simulink model "RM3"  (R2020b)
settings: Solver=ode4  StartTime=0  StopTime=400  FixedStep=0.1  MaxStep=0.1  RelTol=1e-3  EnableMultiTasking=on
undefined symbols (not defined in the file or in its folder): body, constraint, geometry, hydroData, pto
libraries: WECSim_Lib_Body_Elements x2, WECSim_Lib_Constraints x1, WECSim_Lib_Frames x1, WECSim_Lib_PTOs x1
settings Model: Creator=mlawson  LastModifiedBy=akeeste
settings SolverCC: ZeroCrossControl=DisableAll  AlgebraicLoopSolver=LineSearch  AutoInsertRateTranBlk=on
settings DataIOCC: SaveFormat=Array  SaveOutput=off  SaveTime=off  ReturnWorkspaceOutputs=off
settings OptimizationCC: LifeSpan=inf  SimCompilerOptimization=on
settings DebuggingCC: UnderspecifiedInitializationDetection=Classic  MergeDetectMultiDrivingBlocksExec=none  SolverPrmCheckMsg=warning  AllowSymbolicDim=off  StateNameClashWarn=warning  SFUnexpectedBacktrackingDiag=warning  SFNoUnconditionalDefaultTransitionDiag=warning  SFExecutionAtInitializationDiag=none  ArithmeticOperatorsInVariantConditions=warning
settings HardwareCC: ProdBitPerPointer=32  ProdBitPerSizeT=32  ProdBitPerPtrDiffT=32  ProdLargestAtomicFloat=None  ProdIntDivRoundTo=Undefined  ProdEndianess=Unspecified  ProdWordSize=32  ProdHWDeviceType=32-bit Generic
settings ModelReferenceCC: PropagateSignalLabelsOutOfModel=off
settings SFSimCC: SimUseLocalCustomCode=off  CustomCodeUndefinedFunction=UseInterfaceOnly
settings RTWCC: RTWUseLocalCustomCode=off
settings CodeAppCC: StateflowObjectComments=on
settings GRTTargetCC: TargetLangStandard=C89/C90 (ANSI)
settings ConfigComp: CovMetricSettings=dw  CovSaveCumulativeToWorkspaceVar=on  CovSaveSingleToWorkspaceVar=on  CovExternalEMLEnable=off  CovSFcnEnable=off
settings SimscapeCC: SimscapeNormalizeSystem=off
settings ConfigurationSet: Description=SimMechanics 2G
settings ExplorerConfigSet: InternalSimMechanicsExplorerSettings="<ExplorerConfiguration><canonicalview>default</canonicalview><AnimationSetting><BasePlaybackSpeed>1.0</BasePlaybackSpeed><PlaybackSpeedFactor>1.0</PlaybackSpeedFactor></AnimationSetting><TilePanel><TileInfo><Tiles Columns=\"2\" Count=\"4\" Rows=\"2\"><Column Weight=\"0.5\"/><Column Weight=\"0.5\"/><Row Weight=\"0.5\"/><Row Weight=\"0.5\"/><Tile Height=\"1\" Width=\"1\" X=\"0\" Y=\"0\"/><Tile Height=\"1\" Width=\"1\" X=\"0\" Y=\"1\"/><Tile Height=\"1\" Width=\"1\" X=\"1\" Y=\"0\"/><Tile Height=\"1\" Width=\"1\" X=\"1\" Y=\"1\"/></Tiles></TileInfo><SceneInfo><SceneViewer><BGColor><R>0.60000002384185791</R><G>0.60000002384185791</G><B>0.60000002384185791</B></BGColor><Camera><DoPerspective>off</DoPerspective><Position><X>-5.28910957848137908</X><Y>-384.632249072613831</Y><Z>-15.1490561438029978</Z></Position><Center><X>-5.28910957848137908</X><Y>-7.28939721739152446e-06</Y><Z>-15.1490561438029978</Z></Center><Up><X>0</X><Y>-0</Y><Z>1</Z></Up><ViewLimDist>1</ViewLimDist><YLim>29.7178180022969975</YLim><XLim>34.354994301313134</XLim></Camera></SceneViewer><SceneViewer><BGColor><R>0.60000002384185791</R><G>0.60000002384185791</G><B>0.60000002384185791</B></BGColor><Camera><DoPerspective>off</DoPerspective><Position><X>-1.1840554071884688</X><Y>-5.46187101601080105</Y><Z>285.569034477344985</Z></Position><Center><X>-1.1840554071884688</X><Y>-5.46187101601080105</Y><Z>-96.4189878956305506</Z></Center><Up><X>0</X><Y>1</Y><Z>-0</Z></Up><ViewLimDist>1</ViewLimDist><YLim>38.1722158903479212</YLim><XLim>44.1286187054525456</XLim></Camera></SceneViewer><SceneViewer><BGColor><R>0.60000002384185791</R><G>0.60000002384185791</G><B>0.60000002384185791</B></BGColor><Camera><DoPerspective>off</DoPerspective><Position><X>384.632249217085132</X><Y>0.260362946589576594</Y><Z>-15.6955920945191423</Z></Position><Center><X>-7.15773737169911328e-06</X><Y>0.260362946589576594</Y><Z>-15.6955920945191423</Z></Center><Up><X>-0</X><Y>0</Y><Z>1</Z></Up><ViewLimDist>1</ViewLimDist><YLim>30.7766093059417472</YLim><XLim>35.5789996842178908</XLim></Camera></SceneViewer><SceneViewer><BGColor><R>0.60000002384185791</R><G>0.60000002384185791</G><B>0.60000002384185791</B></BGColor><Camera><DoPerspective>off</DoPerspective><Position><X>191.32988391583163</X><Y>-195.842532631356448</Y><Z>177.457736592884231</Z></Position><Center><X>-30.2968327101377994</X><Y>25.7841839946129028</Y><Z>-44.1689800330834714</Z></Center><Up><X>-0.408248290463863073</X><Y>0.408248290463863073</Y><Z>0.816496580927726145</Z></Up><ViewLimDist>1</ViewLimDist><YLim>34.6800041830381574</YLim><XLim>40.0914813458276669</XLim></Camera></SceneViewer></SceneInfo></TilePanel><MechEditorPanel><Cameras/><GfxPanelCameraMap/><VideoCreator><PlaybackSpeedRatio>1.0</PlaybackSpeedRatio><FrameRate>30</FrameRate><VideoFormat>Motion JPEG AVI</VideoFormat><FrameSize>auto</FrameSize></VideoCreator></MechEditorPanel></ExplorerConfiguration>"

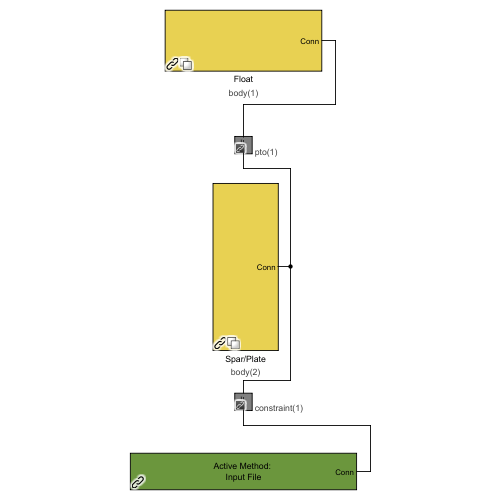
[thumbnail: Simulink's stored preview of the top-level diagram]
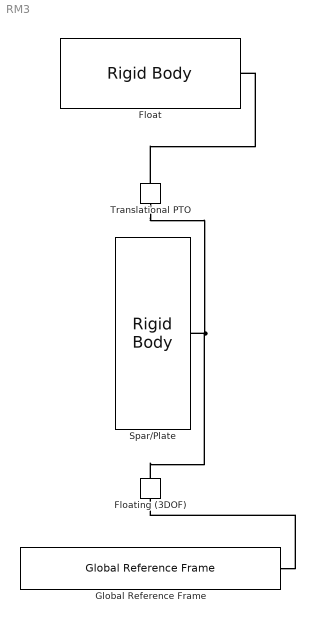
== system RM3 ==
  Float : WECSim_Lib_Body_Elements/Rigid Body  body=body(1)  h5File=hydroData/*.h5  geometryFile=geometry/*.stl  mass=0  inertia=0 0 0  inertiaProducts=0 0 0  nonHydro=0  nonlinearHydro=0  centerGravity=0 0 0  centerBuoyancy=0 0 0  dof=6  volume=0  displacement=0 0 0  axis=0 1 0  angle=0  option=0  cd=0 0 0  ca=0 0 0  area=0 0 0  VME=0  rgME=0 0 0  z=0 0 1
  Floating (3DOF) : WECSim_Lib_Constraints/Floating (3DOF)  constraint=constraint(1)  loc="0  0  0"  displacement=0 0 0  y=0 1 0  z=0 0 1  upperLimitSpecify=off  upperLimitBound=0  upperLimitTransitionRegionWidth=0  upperLimitStiffness=0  upperLimitDamping=0  lowerLimitSpecify=off  lowerLimitBound=0  lowerLimitTransitionRegionWidth=0  lowerLimitStiffness=0  lowerLimitDamping=0
      settings: AttributesFormatString=%<constraint>
  Global Reference Frame : WECSim_Lib_Frames/Global Reference Frame  waves=waves  simu=simu  InputMethod=Input File  InputFile=wecSimInputFile.m  mode=normal  explorer=off  solver=ode4  startTime=0  rampTime=100  endTime=400  dt=0.1  cicEndTime=60  stateSpace=0  WaveClass=regular  height=2.5  period=8  elevationFile=NOT DEFINED  spectrumFile=NOT DEFINED  direction=0  spread=1  spectrumType=NOT DEFINED  phaseSeed=0  option=EqualEnergy
  Spar/Plate : WECSim_Lib_Body_Elements/Rigid Body  body=body(2)  h5File=hydroData/*.h5  geometryFile=geometry/*.stl  mass=0  inertia=0 0 0  inertiaProducts=0 0 0  nonHydro=0  nonlinearHydro=0  centerGravity=0 0 0  centerBuoyancy=0 0 0  dof=6  volume=0  displacement=0 0 0  axis=0 1 0  angle=0  option=0  cd=0 0 0  ca=0 0 0  area=0 0 0  VME=0  rgME=0 0 0  z=0 0 1
  Translational PTO : WECSim_Lib_PTOs/Translational PTO  pto=pto(1)  loc="0  0  0"  stiffness=0  damping=0  equilibriumPosition=0  pretension=0  displacement=0 0 0  y=0 1 0  z=0 0 1  upperLimitSpecify=off  upperLimitBound=0  upperLimitTransitionRegionWidth=0  upperLimitStiffness=0  upperLimitDamping=0  lowerLimitSpecify=off  lowerLimitBound=0  lowerLimitTransitionRegionWidth=0  lowerLimitStiffness=0  lowerLimitDamping=0
      settings: AttributesFormatString=%<pto>
  connections:
  Global Reference Frame/RConn1 -- Floating (3DOF)/LConn1
  Spar/Plate/RConn1 -- Floating (3DOF)/RConn1 -- Translational PTO/RConn1
  Translational PTO/LConn1 -- Float/RConn1
